simulink model "pendulum"  (R2026b)
settings: Solver=ode45  StopTime=Tsim  MaxStep=0.01  RelTol=1e-8  AbsTol=1e-10
InitFcn:
  | pendulum_params;
values from neighbouring files (symbols this model uses):
  a_sw_max = 5    [pendulum_params.m]
  amax = 15    [pendulum_params.m]
  b = 0.15*m    (= 0.045)    [pendulum_params.m]
  beta0 = 0    [pendulum_params.m]
  beta_max = deg2rad(60)    [pendulum_params.m]
  ctrl_on = 1    [pendulum_params.m]
  E_up = 2*m*g*L    (= 5.886)    [pendulum_params.m]
  g = 9.81    [pendulum_params.m]
  J = 0.03    [pendulum_params.m]
  Kb1 = Kb(1)    [pendulum_params.m]
  Kb2 = Kb(2)    [pendulum_params.m]
  Kb3 = Kb(3)    [pendulum_params.m]
  Kb4 = Kb(4)    [pendulum_params.m]
  kb_att = J*wn_att^2    (= 18.75)    [pendulum_params.m]
  kbd_att = 2*zeta_att*wn_att*J    (= 1.2)    [pendulum_params.m]
  kd = 4    [pendulum_params.m]
  kdx = 1.5    [pendulum_params.m]
  kE = 2/m    (= 6.66666666667)    [pendulum_params.m]
  kick_live = 0    [live_pendulum.m]    (also in pendulum_params.m)
  kp = 4    [pendulum_params.m]
  kpx = 1    [pendulum_params.m]
  L = 1.0    (= 1)    [pendulum_params.m]
  l_arm = 0.25    [pendulum_params.m]
  live_on = 0    [pendulum_params.m]
  m = 0.3    [pendulum_params.m]
  M = 1.5    [pendulum_params.m]
  noise_seed = 42    [pendulum_params.m]
  noise_std = dist_on * noise_std    (= 0)    [pendulum_params.m]
  noise_Ts = 0.05    [pendulum_params.m]
  omega0 = 0    [pendulum_params.m]
  p_live = [0; 0]    [live_pendulum.m]    (also in pendulum_params.m)
  phi_catch = deg2rad(50)    [pendulum_params.m]
  phi_release = deg2rad(80)    [pendulum_params.m]
  T_hover = (M + m)*g/2    (= 8.829)    [pendulum_params.m]
  tau_ff = 0.05    [pendulum_params.m]
  tau_m = 0.02    [pendulum_params.m]
  tau_p = 0    [pendulum_params.m]
  theta0 = 0    [pendulum_params.m]
  theta_ref = pi    (= 3.14159265359)    [pendulum_params.m]
  Tmax = 25    [pendulum_params.m]
  v_ref = 0.5    [pendulum_params.m]
  x0 = 0    [pendulum_params.m]
  y0 = 0    [pendulum_params.m]
settings Model: Creator=dawid  LastModifiedBy=dawid
settings OptimizationCC: BlockReduction=off

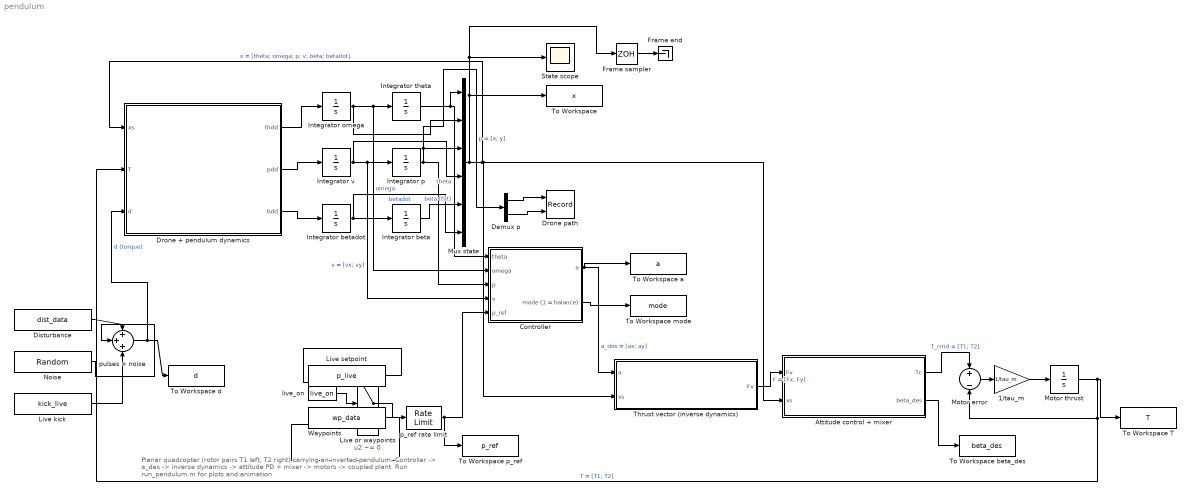
== system pendulum ==
  note: Planar quadcopter (rotor pairs T1 left, T2 right) carrying an inverted pendulum.
      | Controller -> a_des -> inverse dynamics -> attitude PD + mixer -> motors -> coupled plant.
      | Run run_pendulum.m for plots and animation
  1/tau_m : Gain  Gain=1/tau_m
  Attitude control + mixer : MATLAB Function  TreatAsAtomicUnit=on
  Controller : Subsystem
  Demux p : Demux  Outputs=2
  Disturbance : FromWorkspace  VariableName=dist_data  Interpolate=off  OutputAfterFinalValue=Setting to zero
  Drone + pendulum dynamics : MATLAB Function  TreatAsAtomicUnit=on
  Drone path : Record  NumPorts=2.0  FileSettingsInternal="{\"entries\":[{\"content\":{\"excelSettings\":{\"content\":{},\"type\":\"Streamout.ExcelSettings\"},\"parquetSettings\":{\"content\":{},\"type\":\"Streamout.ParquetSettings\"}},\"type\":\"Streamout.FileSettingStorage\",\"uuid\":\"\"}],\"packageUris\":[\"http:\\/\\/schema.mathworks.com\\/mf0\\/streamout_blocks\\/R2020a\"],\"version\":\"1.0\"}"  FrameSettings=[0, 0]  Layout=[1 1]  SignalsInternal="{\"entries\":[{\"content\":{\"signals\":[{\"content\":{\"blockPath\":[],\"dimensions\":[1],\"domain\":\"\",\"lineColor\":\"#a2142f\",\"plots\":[ 1 ],\"port\":1,\"signalID\":1,\"signalName\":\"XY Graph:1\"},\"type\":\"RecordBlkView.Signal\",\"uuid\":\"\"},{\"content\":{\"blockPath\":[],\"dimensions\":[1],\"domain\":\"\",\"lineColor\":\"#139fff\",\"plots\":[ 1 ],\"port\":2,\"signalID\":2,\"signalName\":\"XY Graph:2\"},\"type\":\"RecordBlkView.Signal\",\"uuid\":\"\"}]},\"type\":\"RecordBlkView.InputSignals\",\"uuid\":\"\"}],\"packageUris\":[\"http:\\/\\/schema.mathworks.com\\/mf0\\/streamout_blocks\\/R2020a\"],\"version\":\"1.0\"}"  VisualizationBindings="{\"xyplotplugin\":{\"info\":[{\"series\":[{\"bindingParametersList\":[{\"parameter\":\"X-Axis\",\"signalID\":1,\"signalName\":\"XY Graph:1\"},{\"parameter\":\"Y-Axis\",\"signalID\":2,\"signalName\":\"XY Graph:2\"}],\"seriesID\":0}],\"subplotID\":1}]}}"  CompatibilityTag=XY
  Frame end : Terminator
  Frame sampler : ZeroOrderHold  SampleTime=0.02
  Integrator beta : Integrator  InitialCondition=beta0
  Integrator betadot : Integrator
  Integrator omega : Integrator  InitialCondition=omega0
  Integrator p : Integrator  InitialCondition=[x0; y0]
  Integrator theta : Integrator  InitialCondition=theta0
  Integrator v : Integrator  InitialCondition=[0; 0]
  Live kick : Constant  Value=kick_live  SampleTime=0.02
  Live or waypoints : Switch  Criteria=u2 ~= 0  SaturateOnIntegerOverflow=off  InputSameDT=off
  Live setpoint : Constant  Value=p_live  SampleTime=0.02
  Motor error : Sum  Inputs=+-
  Motor thrust : Integrator  InitialCondition=[T_hover; T_hover]
  Mux state : Mux  Inputs=6
  Noise : RandomNumber  Variance=noise_std^2  Seed=noise_seed  SampleTime=noise_Ts
  State scope : Scope
      settings: TimeSpan=25  ActiveDisplayYMinimum=-8  ActiveDisplayYMaximum=8
  Thrust vector (inverse dynamics) : MATLAB Function  TreatAsAtomicUnit=on
  To Workspace : ToWorkspace  VariableName=x  SaveFormat=Timeseries  SampleTime=-1
  To Workspace T : ToWorkspace  VariableName=T  SaveFormat=Timeseries  SampleTime=-1
  To Workspace a : ToWorkspace  VariableName=a  SaveFormat=Timeseries  SampleTime=-1
  To Workspace beta_des : ToWorkspace  VariableName=beta_des  SaveFormat=Timeseries  SampleTime=-1
  To Workspace d : ToWorkspace  VariableName=d  SaveFormat=Timeseries  SampleTime=-1
  To Workspace mode : ToWorkspace  VariableName=mode  SaveFormat=Timeseries  SampleTime=-1
  To Workspace p_ref : ToWorkspace  VariableName=p_ref  SaveFormat=Timeseries  SampleTime=-1
  Waypoints : FromWorkspace  VariableName=wp_data  Interpolate=off  OutputAfterFinalValue=Holding final value
  live_on : Constant  Value=live_on
  p_ref rate limit : RateLimiter  RisingSlewLimit=v_ref  FallingSlewLimit=-v_ref  SampleTimeMode=inherited
  pulses + noise : Sum  Inputs=+++
  wires:
  Drone + pendulum dynamics/1(thdd) -> Integrator omega/1
  Drone + pendulum dynamics/2(pdd) -> Integrator v/1
  Drone + pendulum dynamics/3(bdd) -> Integrator betadot/1
  Integrator omega/1 -> Integrator theta/1, Controller/2(omega), Mux state/2  "omega"
  Integrator v/1 -> Integrator p/1, Controller/4(v), Mux state/4  "v = [vx; vy]"
  Integrator betadot/1 -> Integrator beta/1, Mux state/6  "betadot"
  Mux state/1 -> Frame sampler/1, State scope/1, To Workspace/1, Attitude control + mixer/2(xs), Thrust vector (inverse dynamics)/2(xs), Drone + pendulum dynamics/1(xs)  "x = [theta; omega; p; v; beta; betadot]"
  Motor thrust/1 -> Drone + pendulum dynamics/2(T), Motor error/2, To Workspace T/1  "T = [T1; T2]"
  pulses + noise/1 -> Drone + pendulum dynamics/3(d), To Workspace d/1  "d (torque)"
  Disturbance/1 -> pulses + noise/1
  Noise/1 -> pulses + noise/2
  Live kick/1 -> pulses + noise/3
  Controller/1(a) -> Thrust vector (inverse dynamics)/1(a), To Workspace a/1  "a_des = [ax; ay]"
  Thrust vector (inverse dynamics)/1(Fv) -> Attitude control + mixer/1(Fv)  "F = [Fx; Fy]"
  Attitude control + mixer/1(Tc) -> Motor error/1  "T_cmd = [T1; T2]"
  Motor error/1 -> 1/tau_m/1
  1/tau_m/1 -> Motor thrust/1
  Attitude control + mixer/2(beta_des) -> To Workspace beta_des/1
  Integrator theta/1 -> Controller/1(theta), Mux state/1  "theta"
  Integrator p/1 -> Mux state/3, Demux p/1, Controller/3(p)  "p = [x; y]"
  Live setpoint/1 -> Live or waypoints/1
  live_on/1 -> Live or waypoints/2
  Waypoints/1 -> Live or waypoints/3
  Live or waypoints/1 -> p_ref rate limit/1
  p_ref rate limit/1 -> Controller/5(p_ref), To Workspace p_ref/1
  Controller/2(mode (1 = balance)) -> To Workspace mode/1
  Integrator beta/1 -> Mux state/5  "beta (tilt)"
  Frame sampler/1 -> Frame end/1
  Demux p/1 -> Drone path/1
  Demux p/2 -> Drone path/2

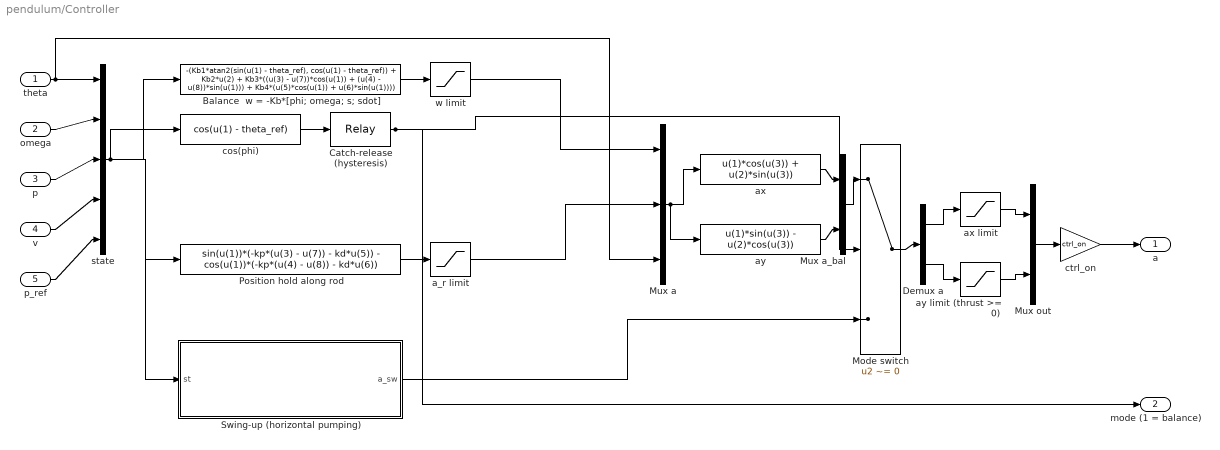
== system pendulum/Controller ==
  theta : Inport
  omega : Inport  Port=2
  p : Inport  Port=3
  v : Inport  Port=4
  p_ref : Inport  Port=5
  Balance  w = -Kb*[phi; omega; s; sdot] : Fcn  Expr=-(Kb1*atan2(sin(u(1) - theta_ref), cos(u(1) - theta_ref)) + Kb2*u(2) + Kb3*((u(3) - u(7))*cos(u(1)) + (u(4) - u(8))*sin(u(1))) + Kb4*(u(5)*cos(u(1)) + u(6)*sin(u(1))))
  Catch-release (hysteresis) : Relay  OnSwitchValue=cos(phi_catch)  OffSwitchValue=cos(phi_release)
  Demux a : Demux  Outputs=2
  Mode switch : Switch  Criteria=u2 ~= 0  SaturateOnIntegerOverflow=off  InputSameDT=off
  Mux a : Mux  Inputs=3
  Mux a_bal : Mux  Inputs=2
  Mux out : Mux  Inputs=2
  Position hold along rod : Fcn  Expr=sin(u(1))*(-kp*(u(3) - u(7)) - kd*u(5)) - cos(u(1))*(-kp*(u(4) - u(8)) - kd*u(6))
  Swing-up (horizontal pumping) : MATLAB Function  TreatAsAtomicUnit=on
  a_r limit : Saturate  UpperLimit=amax  LowerLimit=-amax
  ax : Fcn  Expr=u(1)*cos(u(3)) + u(2)*sin(u(3))
  ax limit : Saturate  UpperLimit=amax  LowerLimit=-amax
  ay : Fcn  Expr=u(1)*sin(u(3)) - u(2)*cos(u(3))
  ay limit (thrust >= 0) : Saturate  UpperLimit=amax  LowerLimit=-g
  cos(phi) : Fcn  Expr=cos(u(1) - theta_ref)
  ctrl_on : Gain  Gain=ctrl_on
  state : Mux  Inputs=5
  w limit : Saturate  UpperLimit=amax  LowerLimit=-amax
  a : Outport
  mode (1 = balance) : Outport  Port=2
  wires:
  theta/1 -> state/1, Mux a/3
  omega/1 -> state/2
  p/1 -> state/3
  v/1 -> state/4
  p_ref/1 -> state/5
  state/1 -> Balance  w = -Kb*[phi; omega; s; sdot]/1, Swing-up (horizontal pumping)/1(st), cos(phi)/1, Position hold along rod/1
  Balance  w = -Kb*[phi; omega; s; sdot]/1 -> w limit/1
  w limit/1 -> Mux a/1
  Position hold along rod/1 -> a_r limit/1
  a_r limit/1 -> Mux a/2
  Mux a/1 -> ax/1, ay/1
  ax/1 -> Mux a_bal/1
  ay/1 -> Mux a_bal/2
  Mux a_bal/1 -> Mode switch/1
  cos(phi)/1 -> Catch-release (hysteresis)/1
  Catch-release (hysteresis)/1 -> Mode switch/2, mode (1 = balance)/1
  Swing-up (horizontal pumping)/1(a_sw) -> Mode switch/3
  Mode switch/1 -> Demux a/1
  Demux a/1 -> ax limit/1
  Demux a/2 -> ay limit (thrust >= 0)/1
  ax limit/1 -> Mux out/1
  ay limit (thrust >= 0)/1 -> Mux out/2
  Mux out/1 -> ctrl_on/1
  ctrl_on/1 -> a/1

== matlab function pendulum/Thrust vector (inverse dynamics) ==
  data: a input size=[2 1]; Fv output size=[2 1]; xs input size=[8 1]; M parameter; m parameter; L parameter; g parameter; b parameter; tau_ff parameter
function Fv = f(a, xs, M, m, L, g, b, tau_ff)
% Predict theta'' for the commanded pivot acceleration a (d unknown -> 0),
% then the mass acceleration, then the force the rod pulls on the drone.
% Evaluated tau_ff ahead: the tilt + motors need that long to deliver it,
% and a late cancellation of the rod pull acts as damping on the swing.
th = xs(1); om = xs(2); bd = xs(8);
thdd0 = (-m*L*(cos(th)*a(1) + sin(th)*a(2)) - m*g*L*sin(th) - b*(om - bd)) / (m*L^2);
th = th + tau_ff*om + 0.5*tau_ff^2*thdd0;
om = om + tau_ff*thdd0;
c = cos(th); s = sin(th);
thdd = (-m*L*(c*a(1) + s*a(2)) - m*g*L*s - b*(om - bd)) / (m*L^2);
qdd  = a + L*(thdd*[c; s] + om^2*[-s; c]);   % mass acceleration
Fv   = M*(a + [0; g]) + m*(qdd + [0; g]);     % drone + what the rod needs

== matlab function pendulum/Drone + pendulum dynamics ==
  data: xs input size=[8 1]; thdd output size=1; T input size=[2 1]; d input size=1; pdd output size=[2 1]; bdd output size=1; M parameter; m parameter; J parameter; L parameter; g parameter; b parameter; l_arm parameter
function [thdd, pdd, bdd] = f(xs, T, d, M, m, J, L, g, b, l_arm)
% Generalised coordinates q = [x; y; theta]; the tilt beta is decoupled
% because the rod is pinned at the drone centre of mass.
th = xs(1); om = xs(2); be = xs(7); bd = xs(8);
c = cos(th); s = sin(th);
F   = T(1) + T(2);              % total thrust along the body axis
tau = l_arm*(T(2) - T(1));      % right pair - left pair -> tilt torque
Mt  = M + m;
fr  = b*(om - bd);              % pivot friction (relative rotation)
MM  = [Mt 0 m*L*c; 0 Mt m*L*s; m*L*c m*L*s m*L^2];
rhs = [-F*sin(be) + m*L*s*om^2;
        F*cos(be) - Mt*g - m*L*c*om^2;
       -m*g*L*s - fr + d];
qdd  = MM \ rhs;
pdd  = qdd(1:2);
thdd = qdd(3);
bdd  = (tau + fr)/J;

== matlab function pendulum/Attitude control + mixer ==
  data: Fv input size=[2 1]; Tc output size=[2 1]; xs input size=[8 1]; beta_des output size=1; kb_att parameter; kbd_att parameter; l_arm parameter; Tmax parameter; beta_max parameter
function [Tc, beta_des] = f(Fv, xs, kb_att, kbd_att, l_arm, Tmax, beta_max)
be = xs(7); bd = xs(8);
beta_des = atan2(-Fv(1), Fv(2));                 % body axis (-sin b, cos b) || Fv
beta_des = min(max(beta_des, -beta_max), beta_max);
e   = atan2(sin(be - beta_des), cos(be - beta_des));
tau = -kb_att*e - kbd_att*bd;                    % attitude PD
% Altitude priority: choose F so the VERTICAL force is right even while the
% tilt is still lagging (a projection onto the axis makes the drone bob,
% and that bobbing pumps energy out of the pendulum).
F   = max(0, Fv(2) / max(cos(be), 0.5));
% Attitude has priority: keep both pairs within [0, Tmax] by limiting F
dT  = min(abs(tau)/(2*l_arm), Tmax/2);
F   = min(max(F, 2*dT), 2*(Tmax - dT));
tau = sign(tau)*2*l_arm*dT;
Tc  = [F/2 - tau/(2*l_arm); F/2 + tau/(2*l_arm)];  % [left pair; right pair]

== matlab function pendulum/Controller/Swing-up (horizontal pumping) ==
  data: st input size=[8 1]; a_sw output size=[2 1]; m parameter; L parameter; g parameter; E_up parameter; kE parameter; a_sw_max parameter; tau_p parameter; kpx parameter; kdx parameter; kp parameter; kd parameter
function a_sw = f(st, m, L, g, E_up, kE, a_sw_max, tau_p, kpx, kdx, kp, kd)
th = st(1); om = st(2);
E   = 0.5*m*L^2*om^2 + m*g*L*(1 - cos(th));
% predict tau_p ahead to cover the attitude + motor lag
omp = om - tau_p*(g/L)*sin(th);
thp = th + tau_p*om;
% dE/dt = -m*L*omega*cos(theta)*ax  ->  pump (or brake) with ax
sw  = omp*cos(thp);
if abs(sw) < 0.05, sw = 0.05; end                     % kick when hanging at rest
ax  = -kE*(E_up - E)*sw;
ax  = min(max(ax, -a_sw_max), a_sw_max) - kpx*(st(3) - st(7)) - kdx*st(5);
ay  = -kp*(st(4) - st(8)) - kd*st(6);                % hold altitude
a_sw = [ax; ay];
